simulink model "Copy_of_RCAM_LQI_with_PID_restored_from_autosave"  (R2024b)
settings: Solver=VariableStepAuto  StartTime=0.0  StopTime=200  RelTol=1e-3
undefined symbols (not defined in the file or in its folder): A_new, B_new, C_lon, D_lon, Ki, Kx, V0
libraries: slpidlib x1
settings Model: Creator=rukky  LastModifiedBy=rukky

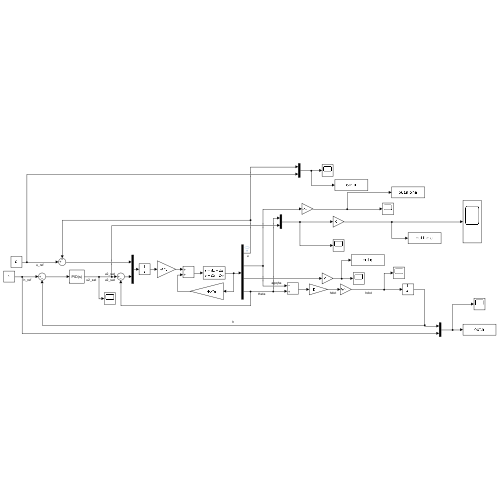
[thumbnail: Simulink's stored preview of the top-level diagram]
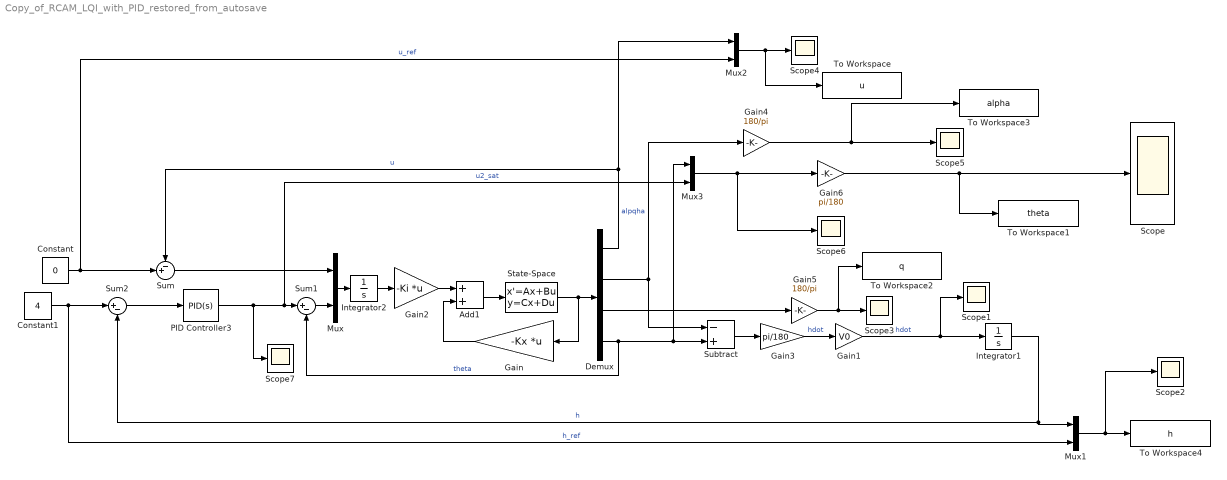
== system Copy_of_RCAM_LQI_with_PID_restored_from_autosave ==
  Add1 : Sum
  Constant : Constant  Value=0
  Constant1 : Constant  Value=4
  Demux : Demux
  Gain : Gain  Gain=-Kx  Multiplication=Matrix(K*u)
  Gain1 : Gain  Gain=V0
  Gain2 : Gain  Gain=-Ki  Multiplication=Matrix(K*u)
  Gain3 : Gain  Gain=pi/180
  Gain4 : Gain  Gain=180/pi
  Gain5 : Gain  Gain=180/pi
  Gain6 : Gain  Gain=pi/180
  Integrator1 : Integrator
  Integrator2 : Integrator
  Mux{,1..3} (4 alike) : Mux  Inputs=2
  PID Controller3 : slpidlib/PID Controller  Controller=PID  Form=Parallel  TimeDomain=Continuous-time  UseExternalTs=off  SampleTime=-1  IntegratorMethod=Forward Euler  FilterMethod=Forward Euler  ControllerParametersSource=internal  P=0.25369448267214  I=0.000355877130606485  UseKiTs=off  D=13.3839088181392  UseExternalDerivativeSource=off  N=19.9247982164299  UseFilter=on  TunerSelectOption=Transfer Function Based (PID Tuner App)  InitialConditionSource=internal  InitialConditionForIntegrator=0  InitialConditionForFilter=0  DifferentiatorICPrevScaledInput=0  ExternalReset=none  TrackingMode=off  Kt=1  LimitOutput=off  SatLimitsSource=internal  UpperSaturationLimit=10  LowerSaturationLimit=-10  LinearizeAsGain=on  AntiWindupMode=clamping  Kb=1  LimitIntegrator=off  UpperIntegratorSaturationLimit=inf  LowerIntegratorSaturationLimit=-inf  POutMin=[]  POutMax=[]  IOutMin=[]  IOutMax=[]  DOutMin=[]  DOutMax=[]  NOutMin=[]  NOutMax=[]  SumOutMin=[]  SumOutMax=[]  SaturationOutMin=[]  SaturationOutMax=[]  PParamMin=[]  PParamMax=[]  IParamMin=[]  IParamMax=[]  DParamMin=[]  DParamMax=[]  NParamMin=[]  NParamMax=[]  KbParamMin=[]  KbParamMax=[]  KtParamMin=[]  KtParamMax=[]  KbOutMin=[]  KbOutMax=[]  KtOutMin=[]  KtOutMax=[]  IntegratorOutMin=[]  IntegratorOutMax=[]  FilterOutMin=[]  FilterOutMax=[]  SumI1OutMin=[]  SumI1OutMax=[]  SumI2OutMin=[]  SumI2OutMax=[]  SumI3OutMin=[]  SumI3OutMax=[]  SumI4OutMin=[]  SumI4OutMax=[]  SumDOutMin=[]  SumDOutMax=[]  DifferentiatorOutMin=[]  DifferentiatorOutMax=[]  FilterDiffOutCoefMin=[]  FilterDiffOutCoefMax=[]  ReciprocalOutMin=[]  ReciprocalOutMax=[]  SumDenOutMin=[]  SumDenOutMax=[]  SumNumOutMin=[]  SumNumOutMax=[]  DivideOutMin=[]  DivideOutMax=[]  UdiffTsProdOutMin=[]  UdiffTsProdOutMax=[]  NTsProdOutMin=[]  NTsProdOutMax=[]  UintegralTsProdOutMin=[]  UintegralTsProdOutMax=[]  UngainTsProdOutMin=[]  UngainTsProdOutMax=[]  ClampingZeroOutDataTypeStr=Inherit: Inherit via back propagation  ClampingZeroOutMin=[]  ClampingZeroOutMax=[]  FilterDenConstantOutDataTypeStr=Inherit: Inherit via back propagation  FilterDenConstantOutMin=[]  FilterDenConstantOutMax=[]  PCopyOutDataTypeStr=Inherit: Inherit via back propagation  PCopyOutMin=[]  PCopyOutMax=[]  NCopyOutDataTypeStr=Inherit: Inherit via back propagation  NCopyOutMin=[]  NCopyOutMax=[]  IntegratorContinuousStateAttributes=''  IntegratorStateMustResolveToSignalObject=off  IntegratorRTWStateStorageClass=Auto  FilterContinuousStateAttributes=''  FilterStateMustResolveToSignalObject=off  FilterRTWStateStorageClass=Auto  ParallelPVariant=InternalParameters  IdealPVariant=Disabled  IVariant=InternalParameters  DVariant=InternalParameters  IntegratorVariant=Continuous  SatVariant=Disabled  AWVariant=Passthrough  PCopyVariant=Disabled  TRVariant=Disabled  FdbkBlocksVariant=Forward  IdealPFdbkVariant=Disabled  SatFdbkVariant=Disabled  DerivativeFilterVariant=ContFilter  NVariant=InternalParameters  NCopyVariant=Disabled  FilterICVariant=InternalICsFilter  IntegratorICVariant=InternalICs  ExternalResetVariant=Disabled  TRSumVariant=Passthrough  SumFdbkVariant=Disabled  SumVariant=Sum_PID  TsampFilterVariant=InternalTs  TsampNgainVariant=Passthrough  TsampIntegralVariant=Disabled_SignalSpec  ExternalSaturationOutDataTypeStr=Inherit: Same as second input  DerivativeSourceVariant=ErrorSignal  PreIntVariant=InternalPreInt
  Scope{,1..7} (8 alike) : Scope
  State-Space : StateSpace  A=A_new  B=B_new  C=C_lon  D=D_lon  InitialCondition=0
  Subtract : Sum  Inputs=-+
  Sum : Sum  Inputs=-+|
  Sum1 : Sum  Inputs=|+-
  Sum2 : Sum  Inputs=|+-
  To Workspace : ToWorkspace  VariableName=u  SaveFormat=Timeseries  SampleTime=-1
  To Workspace1 : ToWorkspace  VariableName=theta  SaveFormat=Timeseries  SampleTime=-1
  To Workspace2 : ToWorkspace  VariableName=q  SaveFormat=Timeseries  SampleTime=-1
  To Workspace3 : ToWorkspace  VariableName=alpha  SaveFormat=Timeseries  SampleTime=-1
  To Workspace4 : ToWorkspace  VariableName=h  SaveFormat=Timeseries  SampleTime=-1
  wires:
  State-Space/1 -> Gain/1, Demux/1
  Demux/1 -> Mux2/1, Sum/1  "u"
  Constant/1 -> Mux2/2, Sum/2  "u_ref"
  Demux/4 -> Sum1/2, Mux3/1, Subtract/2  "theta"
  Demux/3 -> Gain5/1
  Subtract/1 -> Gain3/1
  Gain1/1 -> Scope1/1, Integrator1/1  "hdot"
  Sum2/1 -> PID Controller3/1
  Integrator1/1 -> Mux1/1, Sum2/2  "h"
  Constant1/1 -> Sum2/1, Mux1/2  "h_ref"
  Sum/1 -> Mux/1
  Mux/1 -> Integrator2/1
  Add1/1 -> State-Space/1
  Gain/1 -> Add1/2
  Gain2/1 -> Add1/1
  Sum1/1 -> Mux/2
  Demux/2 -> Subtract/1, Gain4/1  "alpqha"
  Gain3/1 -> Gain1/1  "hdot"
  Mux2/1 -> To Workspace/1, Scope4/1
  Gain4/1 -> Scope5/1, To Workspace3/1
  Integrator2/1 -> Gain2/1
  PID Controller3/1 -> Scope7/1, Mux3/2, Sum1/1  "u2_sat"
  Mux3/1 -> Scope6/1, Gain6/1
  Gain6/1 -> Scope/1, To Workspace1/1
  Gain5/1 -> To Workspace2/1, Scope3/1
  Mux1/1 -> Scope2/1, To Workspace4/1
